simulink model "BLDCSpeedControl_EV_Layout_v2"  (R2024b)
settings: Solver=ode23t  StartTime=0.0  StopTime=0.4  FixedStep=Ts  MaxStep=5e-4  RelTol=1e-3  EnableMultiTasking=on
PreLoadFcn:
  | BLDCSpeedControlData;
PostLoadFcn:
  | % [EV_DAQ_V7_HOOK]
  | try; EV_DAQ_Builder_V7('LoadStop'); catch; end
InitFcn:
  | % [EV_DAQ_V7_HOOK]
  | try; EV_DAQ_Builder_V7('Overrides'); catch ME__daq; fprintf('[DAQ] Overrides error: %s\n', ME__daq.message); end
StartFcn:
  | % [EV_DAQ_V7_HOOK]
  | try; EV_DAQ_Builder_V7('AutoInit'); catch ME__daq; fprintf('[DAQ] Auto-init error: %s\n', ME__daq.message); end
StopFcn:
  | % [EV_DAQ_V7_HOOK]
  | try; EV_DAQ_Builder_V7('PostProcess'); catch ME__daq; fprintf('[DAQ] Post-process error: %s\n', ME__daq.message); end
values from neighbouring files (symbols this model uses):
  cells_parallel = 10    [BLDCSpeedControlData.m]
  cells_series = 13    [BLDCSpeedControlData.m]
  Emax = (I_peak^2 - I_cont^2)*t_peak    (= 1125)    [BLDCSpeedControlData.m]    (also in EV_DAQ_Builder_V7.m = (P.I_peak^2 - P.I_cont^2)*safeBase('t_peak',1))
  Emax_thr = 0.98*Emax    (= 1102.5)    [BLDCSpeedControlData.m]
  emf_max_ev = Ke_ph*w_meas_rpm*2*pi/60    (= 9.33751149817)    [BLDCSpeedControlData.m]
  I_cont = 30    [BLDCSpeedControlData.m]    (also in RunAll.m = rav('I_cont', 30))
  I_peak = 45    [BLDCSpeedControlData.m]    (also in RunAll.m = rav('I_peak', 45))
  Ke_ph = Kt/kappa    (= 0.148611111111)    [BLDCSpeedControlData.m]
  Kii = 100    [BLDCSpeedControlData.m]
  Kiv = 1.5    [BLDCSpeedControlData.m]
  Kiw = 10    [BLDCSpeedControlData.m]    (also in EV_Twin_App.m)
  Kpi = 0.2    [BLDCSpeedControlData.m]
  Kpv = 0.3    [BLDCSpeedControlData.m]
  Kpw = 0.05    [BLDCSpeedControlData.m]    (also in EV_Twin_App.m)
  load_scale = 1    [BLDCSpeedControlData.m]
  p = 4    [BLDCSpeedControlData.m]    (also in EV_BatteryCheck.m = inputParser; EV_DAQ_Builder_V7.m = inputParser; EV_Performance_Audit.m = inputParser; EV_Twin_App.m = r.p)
  r_wheel = 0.25    [BLDCSpeedControlData.m]
  rpm_ramp = 13000    [BLDCSpeedControlData.m]
  rpm_ref = 2950    [BLDCSpeedControlData.m]    (also in RunAll.m = rav('rpm_ref', 2950))
  T_Ifilt = 2e-3    (= 0.002)    [BLDCSpeedControlData.m]
  Ts = 1e-5    (= 1e-05)    [BLDCSpeedControlData.m]    (also in EV_BlackBox_SysID_v2.mat = 0.001; EV_Graphs.m = median(diff(tt));if ~isfinite(Ts)||Ts<=0,Ts=1e-3;end; EV_SysID_Auto.m = 0.001)
  Tsc = 1e-4    (= 0.0001)    [BLDCSpeedControlData.m]
  Vdc = 48    [BLDCSpeedControlData.m]    (also in EV_Twin_App.m)
  Vlim_min = 2    [BLDCSpeedControlData.m]
  wheel_mass = 1.5    [BLDCSpeedControlData.m]
undefined symbols (not defined in the file or in its folder): battery_builder_rtmsupport, DiscIntNeverNeededParam, gcbh
libraries: nesl_utility x17, fl_lib x16, ee_lib x6, eeDiscretePi x2, Batteries2_lib x1, SignalEditorBlockLib x1, eePwmGenerator x1, eeGeneralControl x1
(part 2 of 2)

== system BLDCSpeedControl_EV_Layout_v2/Speed//RPM Controller/Sign ==
  u : Inport
  Constant2 : Constant
  Constant3 : Constant  Value=-1
  Switch : Switch  SaturateOnIntegerOverflow=off  InputSameDT=off
  y : Outport
  wires:
  Constant3/1 -> Switch/3
  Constant2/1 -> Switch/1
  u/1 -> Switch/2
  Switch/1 -> y/1

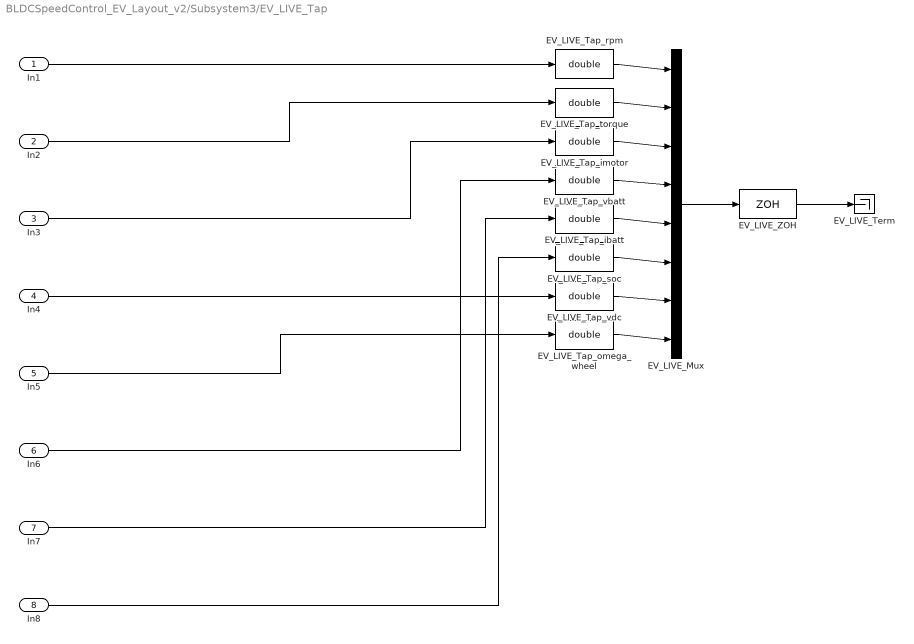
== system BLDCSpeedControl_EV_Layout_v2/Subsystem3/EV_LIVE_Tap ==
  In1 : Inport
  In2 : Inport  Port=2
  In3 : Inport  Port=3
  In4 : Inport  Port=4
  In5 : Inport  Port=5
  In6 : Inport  Port=6
  In7 : Inport  Port=7
  In8 : Inport  Port=8
  EV_LIVE_Mux : Mux  Inputs=8
  EV_LIVE_Tap_ibatt : DataTypeConversion  OutDataTypeStr=double
  EV_LIVE_Tap_imotor : DataTypeConversion  OutDataTypeStr=double
  EV_LIVE_Tap_omega_wheel : DataTypeConversion  OutDataTypeStr=double
  EV_LIVE_Tap_rpm : DataTypeConversion  OutDataTypeStr=double
  EV_LIVE_Tap_soc : DataTypeConversion  OutDataTypeStr=double
  EV_LIVE_Tap_torque : DataTypeConversion  OutDataTypeStr=double
  EV_LIVE_Tap_vbatt : DataTypeConversion  OutDataTypeStr=double
  EV_LIVE_Tap_vdc : DataTypeConversion  OutDataTypeStr=double
  EV_LIVE_Term : Terminator
  EV_LIVE_ZOH : ZeroOrderHold  SampleTime=0.1
  wires:
  EV_LIVE_Mux/1 -> EV_LIVE_ZOH/1
  EV_LIVE_Tap_rpm/1 -> EV_LIVE_Mux/1
  In5/1 -> EV_LIVE_Tap_omega_wheel/1
  EV_LIVE_Tap_imotor/1 -> EV_LIVE_Mux/3
  EV_LIVE_ZOH/1 -> EV_LIVE_Term/1
  EV_LIVE_Tap_torque/1 -> EV_LIVE_Mux/2
  EV_LIVE_Tap_ibatt/1 -> EV_LIVE_Mux/5
  In6/1 -> EV_LIVE_Tap_vbatt/1
  EV_LIVE_Tap_vbatt/1 -> EV_LIVE_Mux/4
  EV_LIVE_Tap_omega_wheel/1 -> EV_LIVE_Mux/8
  EV_LIVE_Tap_soc/1 -> EV_LIVE_Mux/6
  EV_LIVE_Tap_vdc/1 -> EV_LIVE_Mux/7
  In8/1 -> EV_LIVE_Tap_soc/1
  In1/1 -> EV_LIVE_Tap_rpm/1
  In2/1 -> EV_LIVE_Tap_torque/1
  In4/1 -> EV_LIVE_Tap_vdc/1
  In3/1 -> EV_LIVE_Tap_imotor/1
  In7/1 -> EV_LIVE_Tap_ibatt/1

== system BLDCSpeedControl_EV_Layout_v2/Subsystem3/Subsystem ==
  In1 : Inport
  In2 : Inport  Port=2
  In3 : Inport  Port=3
  In4 : Inport  Port=4
  In5 : Inport  Port=5
  In6 : Inport  Port=6
  In7 : Inport  Port=7

== system BLDCSpeedControl_EV_Layout_v2/Subsystem3/Subsystem1 ==
  In1 : Inport
  In2 : Inport  Port=2
  In3 : Inport  Port=3
  In4 : Inport  Port=4
  In5 : Inport  Port=5
  In6 : Inport  Port=6
  In7 : Inport  Port=7
  In8 : Inport  Port=8

== system BLDCSpeedControl_EV_Layout_v2/Subsystem3/Subsystem2 ==
  In1 : Inport
  In2 : Inport  Port=2
  In3 : Inport  Port=3
  In4 : Inport  Port=4
  In5 : Inport  Port=5
  In6 : Inport  Port=6
  In7 : Inport  Port=7
  In8 : Inport  Port=8

== system BLDCSpeedControl_EV_Layout_v2/Sensing w a/Hall sensor/Subsystem ==
  theta : Inport
  Trigonometric Function : Trigonometry  Operator=sincos
  Trigonometric Function2 : Trigonometry  Operator=atan2
  mech->elec : Gain  Gain=p
  rad->deg : Gain  Gain=180/pi  SaturateOnIntegerOverflow=on  OutDataTypeStr=Inherit: Same as input  ParamDataTypeStr=Inherit: Same as input
  deg : Outport  VectorParamsAs1DForOutWhenUnconnected=off
  wires:
  Trigonometric Function2/1 -> rad->deg/1
  Trigonometric Function/1 -> Trigonometric Function2/1
  theta/1 -> mech->elec/1
  rad->deg/1 -> deg/1
  Trigonometric Function/2 -> Trigonometric Function2/2
  mech->elec/1 -> Trigonometric Function/1

== system BLDCSpeedControl_EV_Layout_v2/Speed//RPM Controller/Commutation/Bit concatenate ==
  u : Inport
  Gain : Gain  Gain=[4 2 1]  Multiplication=Matrix(K*u)
  Sum of Elements : Sum  Inputs=+
  y : Outport  VectorParamsAs1DForOutWhenUnconnected=off
  wires:
  u/1 -> Gain/1
  Gain/1 -> Sum of Elements/1
  Sum of Elements/1 -> y/1
